simulink model "s_b4a4x2kf"  (R2016b)
(part 2 of 139)

      mask prompts: io_dir "I/O direction"; io_delay "I/O delay"; sample_period "Sample period"; names "Bitfield names [msb...lsb]"; bitwidths "Bitfield widths"; bin_pts "Bitfield binary pts"; arith_types "Bitfield types, ufix=0, fix=1, bool=2"; sim_port "Provide sim input/output?"; show_format "Print format string?"
      mask help: A 32-bit software-accessible register. Can be divided into bitfields of varying widths and types using the fields in the block mask.
      mask init:
      | swreg_init(gcb)
      settings: AttributesFormatString=1output:uf24.0 = 24 bits
      mask TypeOptions io_dir: To Processor | From Processor
      mask Callback io_dir:
      | mask_enables = get_param(gcb, 'MaskEnables');
      | mask_names = get_param(gcb, 'MaskNames');
      | if strcmp(get_param(gcb, 'io_dir'), 'To Processor'),
      |     mask_enables{ismember(mask_names, 'sample_period')} = 'off';
      | else
      |     mask_enables{ismember(mask_names, 'sample_period')} = 'on';
      | end
      | set_param(gcb, 'MaskEnables', mask_enables);
      mask DialogControl ParameterTabVar0 Prompt: Setup
  xsg : Subsystem  Tag=xps:xsg  AncestorBlock=xps_library/XSG_core_config  mask(xsg core config){hw_sys=SKARAB:xc7vx690t, clk_src=sys_clk, clk_rate=240, sample_period=1, synthesis_tool=XST}
      mask prompts: hw_sys "Hardware Platform"; clk_src "User IP Clock source"; clk_rate "User IP Clock Rate (MHz)"; sample_period "Sample Period"; synthesis_tool "Synthesis Tool:"
      mask help:
      | The XSG Core Config block is used to configure the System Generator design
      | for the casper_xps toolflow. Settings here are used to configure the
      | Xilinx System Generator block parameters automatically, and control toolflow
      | script  execution. It needs to be at the top level of all designs being compiled
      | with the casper_xps toolflow.
      mask init:
      | xps_xsg_conf_mask;
      mask Help: eval('xlWeb([getenv(''MLIB_ROOT''), ''\doc\html\sys_xsg_core_config\sys_xsg_core_config.html''])')
      mask TypeOptions hw_sys: ROACH:sx95t | ROACH:lx110t | ROACH2:sx475t | SNAP:xc7k160t | KC705:xc7k325t | SKARAB:xc7vx690t
      mask Callback hw_sys: xps_xsg_conf_callback
      mask TypeOptions clk_src: sys_clk | aux_clk
      mask Callback clk_src: xps_xsg_conf_callback
      mask Callback clk_rate: xps_xsg_conf_callback
      mask TypeOptions synthesis_tool: Leonardo Spectrum | Synplify | Synplify Pro | XST
      mask Display: fprintf(['MSSGE\n', hw_sys]);
  tag scope: acc_len=global, bf0_gain=global, bf0_id=global, bf0_rst=global, bf0_tx_pkt0=global, bf0_tx_pkt1=global, bf0_tx_pkt2=global, bf0_tx_pkt3=global, bf0_txen=global, bf1_gain=global, bf1_id=global, bf1_rst=global, bf1_tx_pkt0=global, bf1_tx_pkt1=global, bf1_tx_pkt2=global, bf1_tx_pkt3=global, bf1_txen=global, bf_antenna=global, bf_beng=global, bf_data_id=global, bf_stream=global, bf_time_id=global, bf_tvgsel=global, bf_valctrl_bw=global, bf_valctrl_dupl=global, bf_value_bw=global, bf_value_dupl=global, board_id=global, cnt_rst=global, flush=global, gap_size0=global, gap_size1=global, gap_size2=global, gap_size3=global, gbe_rx_bad=global, gbe_rx_overrun=global, gbe_txen=global, go0=global, go1=global, go2=global, go3=global, hmc_pkt_reord_err=global, preproc_snap_dv_mux=global, preproc_snap_stop_mux=global, reord_snap_dv_arm=global, reord_snap_dv_mux=global, snap_reord_stop_sel=global, spead_data=global, spead_fengid=global, spead_freq=global, spead_hdr_err=global, spead_magic_err=global, spead_pad_err=global, spead_pkt_idx=global, spead_pkt_len_err=global, spead_timestamp=global, spead_valid=global, spead_xeng=global, vacc_ld_arm=global, vacc_ld_immediate=global, vacc_ld_time=global, vacc_rst=global, vacctvg_ctr_en=global, vacctvg_data_sel=global, vacctvg_pulse_en=global, vacctvg_reset=global, vacctvg_run=global, vacctvg_sync_sel=global, vacctvg_valid_sel=global, vacctvg_vector_en=global, xeng_tvg_data_sel=global, xeng_tvg_mcnt_sel=global, xeng_tvg_val_sel=global, xengtvg_inj_vector=global
  wires:
  acc_len/1(in_reg) -> Delay21/1(d)
  [gbe_rxvld] -> pipeline76/1(d)
  [gbe_rxdata] -> pipeline75/1(d)
  [gbe_rxeof] -> pipeline77/1(d)
  gbe_porttx/1(in_reg) -> Delay9/1(d)
  gbe_iptx/1(in_reg) -> Delay10/1(d)
  Delay9/1(q) -> [gbe_porttx]
  Delay10/1(q) -> [gbe_iptx]
  board_id/1(in_reg) -> Delay72/1(d)
  control/3(in_cnt_rst) -> pipeline3/1(d)
  control/1(in_vacc_rst) -> pipeline12/1(d)
  control/2(in_status_clr) -> pipeline1/1(d)
  pipeline8/1(q) -> [flasher_en]
  pipeline5/1(q) -> [gbe_txen]
  pipeline2/1(q) -> [gbe_rst]
  edge_detect/1(out) -> [cnt_rst]
  edge_detect3/1(out) -> [clr_status]
  edge_detect2/1(out) -> [vacc_rst]
  edge_detect1/1(out) -> [gbe_debug_rst]
  control/6(in_gbe_debug_rst) -> pipeline4/1(d)
  unpack_feng_hardcoded/1(pkt_start) -> Terminator28/1
  unpack_feng_hardcoded/2(data256) -> pipeline34/1(d)
  unpack_feng_hardcoded/3(valid256) -> Logical6/2, Logical7/2, Logical11/2, Logical10/2, pipeline46/1(d)
  unpack_feng_hardcoded/4(eof256) -> pipeline47/1(d)
  Delay72/1(q) -> [board_id]
  edge_detect5/1(out) -> [reord_snaptrig]
  pipeline13/1(q) -> [reord_snaptrigsel]
  control/8(in_reord_snaptrig) -> pipeline6/1(d)
  vacc_time_msw/3(in_msw) -> Delay19/1(d)
  vacc_time_msw/1(in_arm) -> Delay16/1(d)
  Concat10/1 -> [vacc_ld_time]
  vacc_time_msw/2(in_immediate) -> Delay18/1(d)
  vacc_time_lsw/1(in_lsw) -> Delay20/1(d)
  Delay16/1(q) -> [vacc_ld_arm]
  Delay18/1(q) -> [vacc_ld_immediate]
  Delay19/1(q) -> Concat10/1
  Delay20/1(q) -> Concat10/2
  Delay21/1(q) -> [acc_len]
  spead_time_check/1(lsbzero0) -> speadtime_lsbzero/1(out_spead0)
  pipeline24/1(q) -> [gap_size3]
  pipeline23/1(q) -> [gap_size2]
  pipeline14/1(q) -> [gap_size1]
  pipeline10/1(q) -> [gap_size0]
  pipeline12/1(q) -> edge_detect2/1(in)
  pipeline1/1(q) -> edge_detect3/1(in)
  pipeline3/1(q) -> edge_detect/1(in)
  control/4(in_gbe_rst) -> pipeline2/1(d)
  pipeline4/1(q) -> edge_detect1/1(in)
  pipeline6/1(q) -> edge_detect5/1(in)
  control/5(in_gbe_txen) -> pipeline5/1(d)
  control/7(in_flasher_en) -> pipeline8/1(d)
  control/9(in_reord_snaptrigsel) -> pipeline13/1(d)
  control/10(in_unpack_snapwesel) -> pipeline25/1(d)
  pipeline25/1(q) -> [unpack_snapwesel]
  edge_detect4/1 -> vacc_monitor1/2(new_acc)
  [vacc_err0] -> vacc_monitor1/3(error)
  [cnt_rst] -> vacc_monitor1/1(cnt_rst)
  [pack_txeof0] -> vacc_monitor3/2(eof)
  [pack_err0] -> vacc_monitor3/3(error)
  [cnt_rst] -> vacc_monitor3/1(cnt_rst)
  gapsize/1(in_gap_size) -> Register/1, Relational/2, Delay1/1
  Delay1/1 -> Relational/1
  Register/1 -> pipeline24/1(d), pipeline23/1(d), pipeline14/1(d), pipeline10/1(d)
  bf_config/1(in_data_id) -> pipeline26/1(d)
  bf_config/2(in_time_id) -> pipeline27/1(d)
  bf_control/2(in_stream) -> pipeline29/1(d)
  bf_control/3(in_antenna) -> pipeline30/1(d)
  bf_control/1(in_beng) -> pipeline28/1(d)
  pipeline26/1(q) -> [bf_data_id]
  pipeline27/1(q) -> [bf_time_id]
  pipeline28/1(q) -> [bf_beng]
  pipeline29/1(q) -> [bf_stream]
  pipeline30/1(q) -> [bf_antenna]
  pipeline54/1(q) -> [bf_value_dupl]
  pipeline55/1(q) -> [bf_value_bw]
  bf_value_in0/1(in_dupl) -> pipeline54/1(d)
  bf_value_ctrl/1(in_dupl) -> pipeline32/1(d)
  pipeline32/1(q) -> edge_detect6/1
  pipeline33/1(q) -> edge_detect7/1
  bf_value_ctrl/2(in_bw) -> pipeline33/1(d)
  bf_value_in0/2(in_bw) -> pipeline55/1(d)
  [bfout_valbw0] -> Delay27/1(d)
  [bfout_valbw1] -> Delay26/1(d)
  [bfout_valbw2] -> Delay28/1(d)
  [bfout_valbw3] -> Delay32/1(d)
  Delay27/1(q) -> bf_valout_bw0/1(out_bw0)
  Delay26/1(q) -> bf_valout_bw0/2(out_bw1)
  Delay32/1(q) -> bf_valout_bw1/2(out_bw3)
  Delay28/1(q) -> bf_valout_bw1/1(out_bw2)
  edge_detect6/1 -> [bf_valctrl_dupl]
  edge_detect7/1 -> [bf_valctrl_bw]
  pipeline59/1(q) -> [bf_tvgsel]
  bf_config/3(in_tvg_sel) -> pipeline59/1(d)
  pipeline60/1(q) -> [bf_snap_arm]
  pipeline61/1(q) -> [bf_snap_trig]
  bf_config/4(in_snap_arm) -> pipeline60/1(d)
  bf_config/5(in_snap_trig) -> pipeline61/1(d)
  pipeline65/1(q) -> [vacctvg_sync_sel]
  pipeline62/1(q) -> [vacctvg_valid_sel]
  pipeline64/1(q) -> [vacctvg_reset]
  pipeline66/1(q) -> [vacctvg_data_sel]
  pipeline67/1(q) -> [vacctvg_vector_en]
  pipeline69/1(q) -> [vacctvg_ctr_en]
  pipeline70/1(q) -> [vacctvg_pulse_en]
  pipeline68/1(q) -> [vacctvg_run]
  bf1_config/2(in_beam_id) -> pipeline58/1(d)
  bf1_config/1(in_rst) -> pipeline45/1(d)
  pipeline45/1(q) -> [bf1_rst]
  pipeline58/1(q) -> Convert1/1
  bf1_config/3(in_port) -> pipeline43/1(d)
  pipeline43/1(q) -> [bf1_txport]
  pipeline44/1(q) -> [bf1_txen]
  bf1_config/4(in_txen) -> pipeline44/1(d)
  Convert1/1 -> [bf1_id]
  bf0_config/2(in_beam_id) -> pipeline50/1(d)
  bf0_config/1(in_rst) -> pipeline38/1(d)
  pipeline38/1(q) -> [bf0_rst]
  pipeline50/1(q) -> Convert2/1
  bf0_config/3(in_port) -> pipeline35/1(d)
  pipeline35/1(q) -> [bf0_txport]
  pipeline36/1(q) -> [bf0_txen]
  bf0_config/4(in_txen) -> pipeline36/1(d)
  Convert2/1 -> [bf0_id]
  bf0_ip/1(in_ip) -> pipeline51/1(d)
  pipeline51/1(q) -> [bf0_txip]
  bf1_ip/1(in_ip) -> pipeline52/1(d)
  pipeline52/1(q) -> [bf1_txip]
  bf0_gain/1(in_gain) -> pipeline73/1(d)
  pipeline73/1(q) -> [bf0_gain]
  bf1_gain/1(in_gain) -> pipeline74/1(d)
  pipeline74/1(q) -> [bf1_gain]
  gbe0/1(led_up) -> [gbe_up]
  gbe0/2(led_rx) -> Terminator1/1
  gbe0/3(led_tx) -> Terminator6/1
  gbe0/4(tx_afull) -> Terminator8/1
  gbe0/5(tx_overflow) -> [gbe_tx_over]
  gbe0/6(rx_data) -> [gbe_rxdata]
  gbe0/8(rx_source_ip) -> [gbe_src_ip]
  gbe0/9(rx_source_port) -> [gbe_src_port]
  gbe0/10(rx_end_of_frame) -> [gbe_rxeof]
  gbe0/11(rx_bad_frame) -> [gbe_rx_bad]
  gbe0/12(rx_overrun) -> [gbe_rx_overrun]
  gbe0/14(rx_dest_port) -> [gbe_dest_port]
  gbe0/13(rx_dest_ip) -> [gbe_dest_ip]
  [gbe_rst] -> gbe0/1(rst)
  [gbe_txd] -> gbe0/2(tx_data)
  [gbe_txip] -> gbe0/4(tx_dest_ip)
  [gbe_txport] -> gbe0/5(tx_dest_port)
  [gbe_txeof] -> gbe0/6(tx_end_of_frame)
  Constant3/1 -> gbe0/7(rx_ack)
  Constant4/1 -> gbe0/8(rx_overrun_ack)
  [gbe_debug_rst] -> gbe0/9(debug_rst)
  unpack_feng_hardcoded/13(hdr5_0x1600_DIR) -> pipeline49/1(d)
  unpack_feng_hardcoded/9(hdr_heap_id) -> Terminator2/1
  unpack_feng_hardcoded/10(hdr_heap_size) -> Terminator3/1
  unpack_feng_hardcoded/11(hdr_heap_offset) -> pipeline48/1(d)
  unpack_feng_hardcoded/12(hdr_pkt_len) -> Terminator5/1
  unpack_feng_hardcoded/14(hdr6_0x4101_DIR) -> pipeline53/1(d)
  unpack_feng_hardcoded/16(hdr8_0x4300) -> Terminator31/1
  unpack_feng_hardcoded/15(hdr7_0x4103_DIR) -> pipeline56/1(d)
  pipeline77/1(q) -> unpack_feng_hardcoded/3(pkt_eof)
  pipeline76/1(q) -> unpack_feng_hardcoded/2(pkt_valid)
  pipeline75/1(q) -> unpack_feng_hardcoded/1(pkt_data)
  Concat8/1 -> gbe_mux_bus/1(di)
  [pack_txd1] -> Concat8/2
  [pack_txd0] -> Concat8/1
  Concat11/1 -> gbe_mux_bus/2(validi)
  Concat2/1 -> gbe_mux_bus/3(eofi)
  gbe_mux_bus/5(start) -> bus_expand1/1(bus_in), Delay6/1
  Concat3/1 -> gbe_mux_bus/4(drdy)
  Constant2/1 -> gbe_mux_bus/5(transmit)
  gbe_mux_bus/2(do) -> Delay7/1
  gbe_mux_bus/3(valido) -> Delay17/1
  gbe_mux_bus/4(eofo) -> Delay25/1
  gbe_mux_bus/6(flush) -> [flush]
  [bf0s_d0] -> Concat8/3
  [bf1s_d0] -> Concat8/4
  [pack_txvld0] -> Concat11/1
  [pack_txvld1] -> Concat11/2
  [bf0s_en0] -> Concat11/3
  [bf1s_en0] -> Concat11/4
  [bf0s_eof0] -> Concat2/3
  [bf1s_eof0] -> Concat2/4
  [pack_txeof0] -> Concat2/1
  [pack_txeof1] -> Concat2/2
  [bf0s_pkt_ready0] -> Concat3/3
  [bf1s_pkt_ready0] -> Concat3/4
  [pack_ready1] -> Concat3/2
  [pack_ready0] -> Concat3/1
  [bf0s_d1] -> Concat8/5
  [bf1s_d1] -> Concat8/6
  [bf0s_en1] -> Concat11/5
  [bf1s_en1] -> Concat11/6
  [bf0s_eof1] -> Concat2/5
  [bf1s_eof1] -> Concat2/6
  [bf0s_pkt_ready1] -> Concat3/5
  [bf1s_pkt_ready1] -> Concat3/6
  Delay7/1 -> [gbe_txd]
  Delay17/1 -> [gbe_txvld]
  Delay25/1 -> [gbe_txeof]
  [bf0_txport] -> Mux6/6, Mux6/4
  [bf1_txport] -> Mux6/5, Mux6/7
  [gbe_porttx] -> Mux6/3, Mux6/2
  Mux6/1 -> [gbe_txport]
  gbe_mux_bus/1(input) -> [gbe_ipsel]
  Delay6/1 -> [gbe_txstart]
  Mux5/1 -> [gbe_txip]
  [bf0_txport] -> Mux6/12, Mux6/10
  [bf1_txport] -> Mux6/13, Mux6/11
  [gbe_porttx] -> Mux6/9, Mux6/8
  bus_expand1/12(lsb_out1) -> [bf1_tx_pkt3]
  bus_expand1/1(msb_out12) -> [go0]
  bus_expand1/2(out11) -> [go1]
  bus_expand1/3(out10) -> [bf0_tx_pkt0]
  bus_expand1/4(out9) -> [bf1_tx_pkt0]
  bus_expand1/5(out8) -> [bf0_tx_pkt1]
  bus_expand1/6(out7) -> [bf1_tx_pkt1]
  bus_expand1/7(out6) -> [go2]
  bus_expand1/8(out5) -> [go3]
  bus_expand1/9(out4) -> [bf0_tx_pkt2]
  bus_expand1/10(out3) -> [bf1_tx_pkt2]
  bus_expand1/11(out2) -> [bf0_tx_pkt3]
  [gbe_iptx] -> Concat/1
  [gbe_iptx] -> Concat/2
  [bf0_txip] -> Concat/3
  [bf1_txip] -> Concat/4
  [bf0_txip] -> Concat/5
  [bf1_txip] -> Concat/6
  [gbe_iptx] -> Concat/7
  [gbe_iptx] -> Concat/8
  [bf0_txip] -> Concat/9
  [bf1_txip] -> Concat/10
  [bf0_txip] -> Concat/11
  [bf1_txip] -> Concat/12
  Concat/1 -> bus_addsub/1(a)
  [id2] -> Concat1/9
  [id3] -> Concat1/12
  [id1] -> Concat1/2
  [id0] -> Concat1/1
  [id1] -> Concat1/5
  [id0] -> Concat1/4
  [id3] -> Concat1/8
  [id1] -> Concat1/6
  [id3] -> Concat1/11
  [id2] -> Concat1/10
  [id0] -> Concat1/3
  [id2] -> Concat1/7
  Concat1/1 -> bus_addsub/2(b)
  bus_addsub/1(dout) -> bus_expand/1(bus_in)
  bus_expand/1(msb_out12) -> Mux5/2
  bus_expand/2(out11) -> Mux5/3
  bus_expand/3(out10) -> Mux5/4
  bus_expand/4(out9) -> Mux5/5
  bus_expand/5(out8) -> Mux5/6
  bus_expand/6(out7) -> Mux5/7
  bus_expand/7(out6) -> Mux5/8
  bus_expand/8(out5) -> Mux5/9
  bus_expand/9(out4) -> Mux5/10
  bus_expand/10(out3) -> Mux5/11
  bus_expand/11(out2) -> Mux5/12
  bus_expand/12(lsb_out1) -> Mux5/13
  [pack_txd2] -> Concat8/7
  [pack_txd3] -> Concat8/8
  [pack_txvld2] -> Concat11/7
  [pack_txvld3] -> Concat11/8
  [pack_txeof2] -> Concat2/7
  [pack_txeof3] -> Concat2/8
  [pack_ready2] -> Concat3/7
  [pack_ready3] -> Concat3/8
  [bf0s_d2] -> Concat8/9
  [bf1s_d2] -> Concat8/10
  [bf0s_d3] -> Concat8/11
  [bf1s_d3] -> Concat8/12
  [bf0s_en2] -> Concat11/9
  [bf1s_en2] -> Concat11/10
  [bf0s_en3] -> Concat11/11
  [bf1s_en3] -> Concat11/12
  [bf0s_eof2] -> Concat2/9
  [bf1s_eof2] -> Concat2/10
  [bf0s_eof3] -> Concat2/11
  [bf1s_eof3] -> Concat2/12
  [bf0s_pkt_ready2] -> Concat3/9
  [bf1s_pkt_ready2] -> Concat3/10
  [bf0s_pkt_ready3] -> Concat3/11
  [bf1s_pkt_ready3] -> Concat3/12
  [cnt_rst] -> vacc_monitor2/1(cnt_rst)
  [pack_txeof1] -> vacc_monitor2/2(eof)
  [pack_err1] -> vacc_monitor2/3(error)
  vacc_monitor2/1(pkt_cnt) -> pack_status1/1(out_pkt_cnt)
  vacc_monitor2/2(error_cnt) -> pack_status1/2(out_err_cnt)
  vacc_monitor7/1(pkt_cnt) -> pack_status2/1(out_pkt_cnt)
  vacc_monitor7/2(error_cnt) -> pack_status2/2(out_err_cnt)
  vacc_monitor5/1(pkt_cnt) -> pack_status3/1(out_pkt_cnt)
  vacc_monitor5/2(error_cnt) -> pack_status3/2(out_err_cnt)
  [cnt_rst] -> vacc_monitor7/1(cnt_rst)
  [pack_txeof2] -> vacc_monitor7/2(eof)
  [pack_err2] -> vacc_monitor7/3(error)
  [cnt_rst] -> vacc_monitor5/1(cnt_rst)
  [pack_txeof3] -> vacc_monitor5/2(eof)
  [pack_err3] -> vacc_monitor5/3(error)
  Relational/1 -> Register/2
  [gbe_ipsel] -> Mux5/1
  [gbe_ipsel] -> Mux6/1
  [gbe_txvld] -> gbe0/3(tx_valid)
  gbe0/7(rx_valid) -> [gbe_rxvld]
  vacc_monitor1/1(acc_cnt) -> vacc_status0/1(out_acc_cnt)
  vacc_monitor1/2(error_cnt) -> vacc_status0/2(out_err_cnt)
  [vacc_arm_cnt0] -> vacc_status0/3(out_arm_cnt)
  [vacc_ld_cnt0] -> vacc_status0/4(out_ld_cnt)
  vacc_monitor3/1(pkt_cnt) -> pack_status0/1(out_pkt_cnt)
  vacc_monitor3/2(error_cnt) -> pack_status0/2(out_err_cnt)
  [vacc_rbdone0] -> edge_detect4/1
  edge_detect10/1 -> vacc_monitor4/2(new_acc)
  [vacc_err1] -> vacc_monitor4/3(error)
  [cnt_rst] -> vacc_monitor4/1(cnt_rst)
  vacc_monitor4/1(acc_cnt) -> vacc_status1/1(out_acc_cnt)
  vacc_monitor4/2(error_cnt) -> vacc_status1/2(out_err_cnt)
  [vacc_arm_cnt1] -> vacc_status1/3(out_arm_cnt)
  [vacc_ld_cnt1] -> vacc_status1/4(out_ld_cnt)
  [vacc_rbdone1] -> edge_detect10/1
  edge_detect12/1 -> vacc_monitor6/2(new_acc)
  [vacc_err2] -> vacc_monitor6/3(error)
  [cnt_rst] -> vacc_monitor6/1(cnt_rst)
  vacc_monitor6/1(acc_cnt) -> vacc_status2/1(out_acc_cnt)
  vacc_monitor6/2(error_cnt) -> vacc_status2/2(out_err_cnt)
  [vacc_arm_cnt2] -> vacc_status2/3(out_arm_cnt)
  [vacc_ld_cnt2] -> vacc_status2/4(out_ld_cnt)
  [vacc_rbdone2] -> edge_detect12/1
  edge_detect11/1 -> vacc_monitor8/2(new_acc)
  [vacc_err3] -> vacc_monitor8/3(error)
  [cnt_rst] -> vacc_monitor8/1(cnt_rst)
  vacc_monitor8/1(acc_cnt) -> vacc_status3/1(out_acc_cnt)
  vacc_monitor8/2(error_cnt) -> vacc_status3/2(out_err_cnt)
  [vacc_arm_cnt3] -> vacc_status3/3(out_arm_cnt)
  [vacc_ld_cnt3] -> vacc_status3/4(out_ld_cnt)
  [vacc_rbdone3] -> edge_detect11/1
  miss_cnt0/4(timeout_errctr) -> reord_status0/4(out_timeout_err_cnt)
  miss_cnt0/2(spectr_cnt) -> reord_status0/2(out_sync_cnt)
  miss_cnt0/5(pktdisc_errctr) -> reord_status0/5(out_discard_err_cnt)
  miss_cnt0/3(recv_errctr) -> reord_status0/3(out_missed_err_cnt)
  miss_cnt0/1(last_missed_ant) -> reord_status0/1(out_last_missed_ant)
  miss_cnt1/3(recv_errctr) -> reord_status1/3(out_missed_err_cnt)
  miss_cnt1/4(timeout_errctr) -> reord_status1/4(out_timeout_err_cnt)
  miss_cnt1/5(pktdisc_errctr) -> reord_status1/5(out_discard_err_cnt)
  miss_cnt1/2(spectr_cnt) -> reord_status1/2(out_sync_cnt)
  miss_cnt1/1(last_missed_ant) -> reord_status1/1(out_last_missed_ant)
  miss_cnt2/4(timeout_errctr) -> reord_status2/4(out_timeout_err_cnt)
  miss_cnt2/3(recv_errctr) -> reord_status2/3(out_missed_err_cnt)
  miss_cnt2/1(last_missed_ant) -> reord_status2/1(out_last_missed_ant)
  miss_cnt2/5(pktdisc_errctr) -> reord_status2/5(out_discard_err_cnt)
  miss_cnt2/2(spectr_cnt) -> reord_status2/2(out_sync_cnt)
  miss_cnt3/2(spectr_cnt) -> reord_status3/2(out_sync_cnt)
  miss_cnt3/1(last_missed_ant) -> reord_status3/1(out_last_missed_ant)
  miss_cnt3/3(recv_errctr) -> reord_status3/3(out_missed_err_cnt)
  miss_cnt3/4(timeout_errctr) -> reord_status3/4(out_timeout_err_cnt)
  miss_cnt3/5(pktdisc_errctr) -> reord_status3/5(out_discard_err_cnt)
  unpack_feng_hardcoded/5(magic_error) -> Logical6/1
  unpack_feng_hardcoded/6(hdr_error) -> Logical7/1
  unpack_feng_hardcoded/7(pad_error) -> Logical10/1
  unpack_feng_hardcoded/8(pkt_len_err) -> Logical11/1
  Logical6/1 -> [spead_magic_err]
  Logical7/1 -> [spead_hdr_err]
  Logical10/1 -> [spead_pad_err]
  Logical11/1 -> [spead_pkt_len_err]
  pipeline48/1(q) -> hmc_pkt_reord/6(heap_offset)
  pipeline34/1(q) -> hmc_pkt_reord/1(data_in)
  pipeline49/1(q) -> hmc_pkt_reord/4(spead_time48)
  pipeline53/1(q) -> hmc_pkt_reord/5(spead_fengid)
  pipeline56/1(q) -> hmc_pkt_reord/7(freq_base)
  pipeline46/1(q) -> hmc_pkt_reord/2(valid_in)
  pipeline47/1(q) -> [spead_eof], hmc_pkt_reord/3(eof_in)
  [spead_pkt_len_err] -> Subsystem2/5(in3)
  [spead_pad_err] -> Subsystem2/4(in2)
  Subsystem2/5(out4) -> spead_status/5(out_pkt_cnt)
  Subsystem2/4(out3) -> spead_status/4(out_pkt_len_err_cnt)
  Subsystem2/3(out2) -> spead_status/3(out_pad_err_cnt)
  Subsystem2/2(out1) -> spead_status/2(out_header_err_cnt)
  Subsystem2/1(out0) -> spead_status/1(out_magic_err_cnt)
  [cnt_rst] -> Subsystem2/1(rst)
  [spead_magic_err] -> Subsystem2/2(in0)
  [spead_hdr_err] -> Subsystem2/3(in1)
  [spead_eof] -> Subsystem2/6(in4)
  [cnt_rst] -> Subsystem/1(rst)
  Subsystem/1(Out1) -> bf0_status0/1(out_pkt_cnt)
  Subsystem/2(Out2) -> bf0_status0/2(out_of_err_cnt)
  [bf0s_eof0] -> Subsystem/2(in0)
  [bf0s_of0] -> Subsystem/3(in1)
  Subsystem3/1(Out1) -> bf0_status1/1(out_pkt_cnt)
  Subsystem3/2(Out2) -> bf0_status1/2(out_of_err_cnt)
  [cnt_rst] -> Subsystem3/1(rst)
  [bf0s_eof1] -> Subsystem3/2(in0)
  [bf0s_of1] -> Subsystem3/3(in1)
  Subsystem4/1(Out1) -> bf0_status2/1(out_pkt_cnt)
  Subsystem4/2(Out2) -> bf0_status2/2(out_of_err_cnt)
  Subsystem5/1(Out1) -> bf0_status3/1(out_pkt_cnt)
  Subsystem5/2(Out2) -> bf0_status3/2(out_of_err_cnt)
  Subsystem6/1(Out1) -> bf1_status0/1(out_pkt_cnt)
  Subsystem6/2(Out2) -> bf1_status0/2(out_of_err_cnt)
  Subsystem7/1(Out1) -> bf1_status1/1(out_pkt_cnt)
  Subsystem7/2(Out2) -> bf1_status1/2(out_of_err_cnt)
  Subsystem8/1(Out1) -> bf1_status2/1(out_pkt_cnt)
  Subsystem8/2(Out2) -> bf1_status2/2(out_of_err_cnt)
  Subsystem9/1(Out1) -> bf1_status3/1(out_pkt_cnt)
  Subsystem9/2(Out2) -> bf1_status3/2(out_of_err_cnt)
  [bf0s_of2] -> Subsystem4/3(in1)
  [bf0s_eof2] -> Subsystem4/2(in0)
  [cnt_rst] -> Subsystem9/1(rst)
  [cnt_rst] -> Subsystem8/1(rst)
  [cnt_rst] -> Subsystem7/1(rst)
  [cnt_rst] -> Subsystem6/1(rst)
  [cnt_rst] -> Subsystem5/1(rst)
  [cnt_rst] -> Subsystem4/1(rst)
  [bf1s_eof2] -> Subsystem8/2(in0)
  [bf1s_eof3] -> Subsystem9/2(in0)
  [bf1s_of0] -> Subsystem6/3(in1)
  [bf0s_eof3] -> Subsystem5/2(in0)
  [bf0s_of3] -> Subsystem5/3(in1)
  [bf1s_eof0] -> Subsystem6/2(in0)
  [bf1s_eof1] -> Subsystem7/2(in0)
  [bf1s_of1] -> Subsystem7/3(in1)
  [bf1s_of2] -> Subsystem8/3(in1)
  [bf1s_of3] -> Subsystem9/3(in1)
  tvg_control/9(in_reord_snap_dv_mux) -> pipeline7/1(d)
  tvg_control/11(in_reord_snap_dv_arm) -> pipeline11/1(d)
  tvg_control/12(in_preproc_snap_dv_mux) -> pipeline15/1(d)
  tvg_control/13(in_snap_reord_stop_sel) -> pipeline16/1(d)
  pipeline7/1(q) -> [reord_snap_dv_mux]
  pipeline11/1(q) -> [reord_snap_dv_arm]
  pipeline15/1(q) -> [preproc_snap_dv_mux]
  pipeline16/1(q) -> [snap_reord_stop_sel]
  pipeline9/1(q) -> [xeng_tvg_data_sel]
  tvg_control/10(in_xeng_tvg_data_sel) -> pipeline9/1(d)
  tvg_control/14(in_xeng_tvg_val_sel) -> pipeline17/1(d)
  tvg_control/15(in_xeng_tvg_inj_vector) -> pipeline18/1(d)
  tvg_control/16(in_xeng_tvg_mcnt_sel) -> pipeline19/1(d)
  pipeline17/1(q) -> [xeng_tvg_val_sel]
  pipeline18/1(q) -> [xengtvg_inj_vector]
  pipeline19/1(q) -> [xeng_tvg_mcnt_sel]
  tvg_control/2(in_vacc_tvg_sync_sel) -> pipeline65/1(d)
  tvg_control/3(in_vacc_tvg_valid_sel) -> pipeline62/1(d)
  tvg_control/4(in_vacc_tvg_data_sel) -> pipeline66/1(d)
  tvg_control/5(in_vacc_tvg_reset) -> pipeline64/1(d)
  tvg_control/6(in_vacc_tvg_ctr_en) -> pipeline69/1(d)
  tvg_control/7(in_vacc_tvg_vector_en) -> pipeline67/1(d)
  tvg_control/8(in_vacc_tvg_run) -> pipeline68/1(d)
  tvg_control/1(in_vacc_tvg_pulse_en) -> pipeline70/1(d)
  tvg_control/17(in_preproc_snap_stop_mux) -> pipeline20/1(d)
  pipeline20/1(q) -> [preproc_snap_stop_mux]
  [vacc_time0] -> pipeline/1(d)
  [vacc_time1] -> pipeline21/1(d)
  [vacc_time2] -> pipeline22/1(d)
  [vacc_time3] -> pipeline31/1(d)
  pipeline/1(q) -> vacc_timestamp0/1(out_vacc_timestamp)
  pipeline21/1(q) -> vacc_timestamp1/1(out_vacc_timestamp)
  pipeline22/1(q) -> vacc_timestamp2/1(out_vacc_timestamp)
  pipeline31/1(q) -> vacc_timestamp3/1(out_vacc_timestamp)
  hmc_pkt_reord/1(data_out) -> [spead_data]
  hmc_pkt_reord/2(valid) -> [spead_valid]
  hmc_pkt_reord/3(timestamp) -> [spead_timestamp]
  hmc_pkt_reord/4(src_feng) -> [spead_fengid]
  hmc_pkt_reord/5(freq_this_eng) -> [spead_freq]
  hmc_pkt_reord/6(dest_xeng_this_brd) -> [spead_xeng]
  hmc_pkt_reord/8(err) -> [hmc_pkt_reord_err]
  [board_id] -> hmc_pkt_reord/8(board_id)
  hmc_pkt_reord/7(pkt_idx) -> [spead_pkt_idx]
  [cnt_rst] -> Subsystem1/1(rst)
  [hmc_pkt_reord_err] -> Subsystem1/2(in0)
  Subsystem1/1(Out1) -> hmc_pkt_reord_status/1(out_err_cnt)
  pipeline37/1(q) -> [snp_hmc_pkt_mux_we_sel]
  tvg_control/18(in_snap_hmc_pkt_mux_we_sel) -> pipeline37/1(d)
  [gbe_ipsel] -> Delay81/1
  [gbe_txeof] -> snap_pack_mux/2(in_eof)
  Delay81/1 -> snap_pack_mux/1(in_input_select)
  [gbe_txvld] -> snap_pack_mux/52(we)
  [go3] -> snap_pack_mux/6(in_go3)
  [go2] -> snap_pack_mux/5(in_go2)
  [go1] -> snap_pack_mux/4(in_go1)
  [go0] -> snap_pack_mux/3(in_go0)
  [bf0_tx_pkt0] -> snap_pack_mux/7(in_bf0_tx_pkt0)
  [bf0_tx_pkt1] -> snap_pack_mux/8(in_bf0_tx_pkt1)
  [bf0_tx_pkt2] -> snap_pack_mux/9(in_bf0_tx_pkt2)
  [bf0_tx_pkt3] -> snap_pack_mux/10(in_bf0_tx_pkt3)
  [bf1_tx_pkt0] -> snap_pack_mux/11(in_bf1_tx_pkt0)
  [bf1_tx_pkt1] -> snap_pack_mux/12(in_bf1_tx_pkt1)
  [bf1_tx_pkt2] -> snap_pack_mux/13(in_bf1_tx_pkt2)
  [bf1_tx_pkt3] -> snap_pack_mux/14(in_bf1_tx_pkt3)
  [pack_ready0] -> snap_pack_mux/15(in_rdy0)
  [pack_ready1] -> snap_pack_mux/16(in_rdy1)
  [pack_ready2] -> snap_pack_mux/17(in_rdy2)
  [pack_ready3] -> snap_pack_mux/18(in_rdy3)
  [bf0s_pkt_ready0] -> snap_pack_mux/19(in_bf0_rdy0)
  [bf0s_pkt_ready1] -> snap_pack_mux/20(in_bf0_rdy1)
  [bf0s_pkt_ready2] -> snap_pack_mux/21(in_bf0_rdy2)
  [bf0s_pkt_ready3] -> snap_pack_mux/22(in_bf0_rdy3)
  [bf1s_pkt_ready0] -> snap_pack_mux/23(in_bf1_rdy0)
  [bf1s_pkt_ready1] -> snap_pack_mux/24(in_bf1_rdy1)
  [bf1s_pkt_ready2] -> snap_pack_mux/25(in_bf1_rdy2)
  [bf1s_pkt_ready3] -> snap_pack_mux/26(in_bf1_rdy3)
  [bf1s_en0] -> snap_pack_mux/35(in_bf1_vld0)
  [pack_txvld3] -> snap_pack_mux/30(in_vld3)
  [pack_txvld0] -> snap_pack_mux/27(in_vld0)
  [bf1s_en3] -> snap_pack_mux/38(in_bf1_vld3)
  [bf0s_en1] -> snap_pack_mux/32(in_bf0_vld1)
  [pack_txvld1] -> snap_pack_mux/28(in_vld1)
  [bf0s_en0] -> snap_pack_mux/31(in_bf0_vld0)
  [bf0s_en3] -> snap_pack_mux/34(in_bf0_vld3)
  [pack_txvld2] -> snap_pack_mux/29(in_vld2)
  [bf0s_en2] -> snap_pack_mux/33(in_bf0_vld2)
  [bf1s_en2] -> snap_pack_mux/37(in_bf1_vld2)
  [bf1s_en1] -> snap_pack_mux/36(in_bf1_vld1)
  [bf1s_eof3] -> snap_pack_mux/50(in_bf1_eof3)
  [bf0s_eof2] -> snap_pack_mux/45(in_bf0_eof2)
  [bf0s_eof0] -> snap_pack_mux/43(in_bf0_eof0)
  [pack_txeof3] -> snap_pack_mux/42(in_eof3)
  [bf1s_eof1] -> snap_pack_mux/48(in_bf1_eof1)
  [pack_txeof0] -> snap_pack_mux/39(in_eof0)
  [bf0s_eof1] -> snap_pack_mux/44(in_bf0_eof1)
  [pack_txeof2] -> snap_pack_mux/41(in_eof2)
  [bf0s_eof3] -> snap_pack_mux/46(in_bf0_eof3)
  [bf1s_eof2] -> snap_pack_mux/49(in_bf1_eof2)
  [bf1s_eof0] -> snap_pack_mux/47(in_bf1_eof0)
  [pack_txeof1] -> snap_pack_mux/40(in_eof1)
  [gbe_txeof] -> snap_pack_mux/53(trig)
  [gbe_txip] -> Slice/1
  Slice/1 -> snap_pack_mux/51(in_ip)
